simulink model "tractor_mu"  (R2022b)
settings: Solver=FixedStepDiscrete  StartTime=0.0  StopTime=20  FixedStep=0.001  RelTol=1e-3
model workspace (MAT data in the model file):
  P : object (value not decoded)
  w_2 : Simulink.Parameter (value not decoded)
undefined symbols (not defined in the file): A, a, B, b, C, D, DiscIntNeverNeededParam, Iz, K, k1, K1, k2, K2, L1, L2, m, magnitude, Phi, Sample_time, Steer_Ratio
libraries: simulink x26, slpidlib x13, Solver_SF x1, dsparch4 x1
(part 2 of 7)

== system tractor_mu/垂直载荷估算 ==
  ax : Inport
  ay : Inport  Port=2
  roll : Inport  Port=3
  pitch : Inport  Port=4
  MATLAB Function : MATLAB Function  TreatAsAtomicUnit=on
  MATLAB Function1 : MATLAB Function  Commented=on  TreatAsAtomicUnit=on
  MATLAB Function2 : MATLAB Function  Commented=on  TreatAsAtomicUnit=on
  Mux : Mux
  axay : Scope  Commented=on  NumInputPorts=4
  原方法 : Scope  Commented=on  NumInputPorts=4
  Fz1 : Outport
  Fz2 : Outport  Port=2
  Fz3 : Outport  Port=3
  Fz4 : Outport  Port=4
  Fz : Outport  Port=5
  wires:
  ax/1 -> MATLAB Function2/1(ax), MATLAB Function1/1(ax), MATLAB Function/1(ax)
  ay/1 -> MATLAB Function2/2(ay), MATLAB Function1/2(ay), MATLAB Function/2(ay)
  MATLAB Function/2(Fz2) -> Mux/2, Fz2/1
  MATLAB Function/3(Fz3) -> Mux/3, Fz3/1
  MATLAB Function/4(Fz4) -> Mux/4, Fz4/1
  pitch/1 -> MATLAB Function2/3(alpha), MATLAB Function1/3(alpha), MATLAB Function/3(alpha)
  roll/1 -> MATLAB Function2/4(belta), MATLAB Function1/4(belta), MATLAB Function/4(belta)
  MATLAB Function1/1(Fz1) -> axay/1
  MATLAB Function1/2(Fz2) -> axay/2
  MATLAB Function1/3(Fz3) -> axay/3
  MATLAB Function1/4(Fz4) -> axay/4
  MATLAB Function2/1(Fz1) -> 原方法/1
  MATLAB Function2/2(Fz2) -> 原方法/2
  MATLAB Function2/3(Fz3) -> 原方法/3
  MATLAB Function2/4(Fz4) -> 原方法/4
  MATLAB Function/1(Fz1) -> Mux/1, Fz1/1
  Mux/1 -> Fz/1

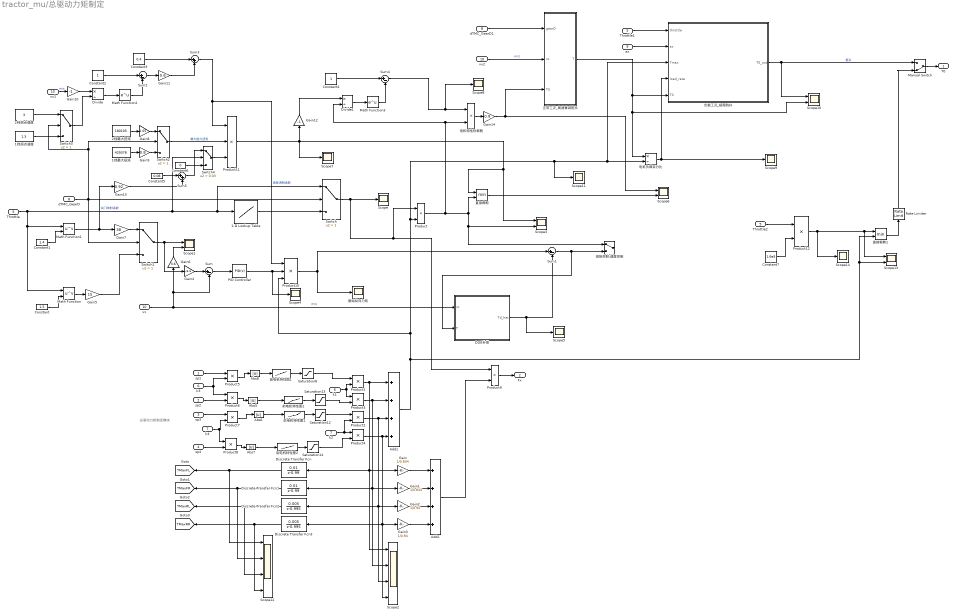
== system tractor_mu/总驱动力矩制定 ==
  note: 总驱动力矩制定模块
  sp1 : Inport
  sp2 : Inport  Port=2
  sp3 : Inport  Port=3
  sp4 : Inport  Port=4
  Throttle : Inport  Port=5
  k1 : Inport  Port=6
  k2 : Inport  Port=7
  dTMC_GearD : Inport  Port=8
  ax : Inport  Port=9
  vx : Inport  Port=10
  1-D Lookup Table : Lookup_n-D  NumberOfTableDimensions=1  BreakpointsForDimension1=[0 0.1 0.2 0.3 0.4 0.5 0.6 0.7 0.8 0.9 1]  Table=[0 0.02 0.04 0.09 0.14 0.23 0.32 0.46 0.6 0.8 1]  InternalRulePriority=Speed  RndMeth=Simplest
  1档拐点速度 : Constant  Value=1.5
  1档最大扭矩 : Constant  Value=429378
  2档拐点速度 : Constant  Value=3
  2档最大扭矩 : Constant  Value=180105
  Abs{5..8} (4 alike) : Abs  SaturateOnIntegerOverflow=off
  Add1 : Sum  Inputs=++++
  Add2 : Sum  Inputs=++++
  Constant : Constant  Value=1.5
  Constant1 : Constant  Value=1.4
  Constant2 : Constant
  Constant3 : Constant  Value=0.4
  Constant4 : Constant
  Constant5 : Constant  Value=0.08
  Constant6 : Constant  Value=0
  Constant7 : Constant  Value=1.6e5
  DOB补偿 : Subsystem
  Discrete Transfer Fcn : DiscreteTransferFcn  Numerator=[0.01]  Denominator=[1 -0.99]
  Discrete Transfer Fcn1 : DiscreteTransferFcn  Numerator=[0.01]  Denominator=[1 -0.99]
  Discrete Transfer Fcn2 : DiscreteTransferFcn  Numerator=[0.005]  Denominator=[1 -0.995]
  Discrete Transfer Fcn3 : DiscreteTransferFcn  Numerator=[0.005]  Denominator=[1 -0.995]
  Divide : Product  Inputs=*/
  Divide1 : Product  Inputs=*/
  Gain : Gain  Gain=1/0.834
  Gain1 : Gain  Gain=1/0.834
  Gain10 : Gain  Gain=-1
  Gain11 : Gain  Gain=0.6
  Gain12 : Gain  Gain=-1
  Gain13 : Gain  Gain=0.92
  Gain14 : Gain  Gain=0.9
  Gain2 : Gain  Gain=1/0.94
  Gain3 : Gain  Gain=1/0.94
  Gain4 : Gain  Gain=1/3.6
  Gain5 : Gain  Gain=15
  Gain6 : Gain  Gain=3.6
  Gain7 : Gain  Gain=38
  Gain8 : Gain  Gain=0.65
  Gain9 : Gain  Gain=0.8
  Manual Switch : ManualSwitch  CurrentSetting=0
  Math Function : Math  Operator=pow
  Math Function1 : Math  Operator=pow
  Math Function2 : Math
  Math Function3 : Math
  PID Controller : slpidlib/PID Controller  Controller=PID  Form=Parallel  TimeDomain=Discrete-time  UseExternalTs=off  SampleTime=-1  IntegratorMethod=Forward Euler  FilterMethod=Forward Euler  ControllerParametersSource=internal  P=0.3  I=0.1  UseKiTs=off  D=0  N=100  UseFilter=on  TunerSelectOption=Transfer Function Based (PID Tuner App)  InitialConditionSource=internal  InitialConditionForIntegrator=0  InitialConditionForFilter=0  DifferentiatorICPrevScaledInput=0  ExternalReset=none  TrackingMode=off  Kt=1  LimitOutput=on  SatLimitsSource=internal  UpperSaturationLimit=1  LowerSaturationLimit=0  LinearizeAsGain=on  AntiWindupMode=none  Kb=1  LimitIntegrator=off  UpperIntegratorSaturationLimit=inf  LowerIntegratorSaturationLimit=-inf  POutMin=[]  POutMax=[]  IOutMin=[]  IOutMax=[]  DOutMin=[]  DOutMax=[]  NOutMin=[]  NOutMax=[]  SumOutMin=[]  SumOutMax=[]  SaturationOutMin=[]  SaturationOutMax=[]  PParamMin=[]  PParamMax=[]  IParamMin=[]  IParamMax=[]  DParamMin=[]  DParamMax=[]  NParamMin=[]  NParamMax=[]  KbParamMin=[]  KbParamMax=[]  KtParamMin=[]  KtParamMax=[]  KbOutMin=[]  KbOutMax=[]  KtOutMin=[]  KtOutMax=[]  IntegratorOutMin=[]  IntegratorOutMax=[]  FilterOutMin=[]  FilterOutMax=[]  SumI1OutMin=[]  SumI1OutMax=[]  SumI2OutMin=[]  SumI2OutMax=[]  SumI3OutMin=[]  SumI3OutMax=[]  SumI4OutMin=[]  SumI4OutMax=[]  SumDOutMin=[]  SumDOutMax=[]  DifferentiatorOutMin=[]  DifferentiatorOutMax=[]  FilterDiffOutCoefMin=[]  FilterDiffOutCoefMax=[]  ReciprocalOutMin=[]  ReciprocalOutMax=[]  SumDenOutMin=[]  SumDenOutMax=[]  SumNumOutMin=[]  SumNumOutMax=[]  DivideOutMin=[]  DivideOutMax=[]  UdiffTsProdOutMin=[]  UdiffTsProdOutMax=[]  NTsProdOutMin=[]  NTsProdOutMax=[]  UintegralTsProdOutMin=[]  UintegralTsProdOutMax=[]  UngainTsProdOutMin=[]  UngainTsProdOutMax=[]  ClampingZeroOutDataTypeStr=Inherit: Inherit via back propagation  ClampingZeroOutMin=[]  ClampingZeroOutMax=[]  FilterDenConstantOutDataTypeStr=Inherit: Inherit via back propagation  FilterDenConstantOutMin=[]  FilterDenConstantOutMax=[]  PCopyOutDataTypeStr=Inherit: Inherit via back propagation  PCopyOutMin=[]  PCopyOutMax=[]  NCopyOutDataTypeStr=Inherit: Inherit via back propagation  NCopyOutMin=[]  NCopyOutMax=[]  IntegratorContinuousStateAttributes=''  IntegratorStateMustResolveToSignalObject=off  IntegratorRTWStateStorageClass=Auto  FilterContinuousStateAttributes=''  FilterStateMustResolveToSignalObject=off  FilterRTWStateStorageClass=Auto  ParallelPVariant=InternalParameters  IdealPVariant=Disabled  IVariant=InternalParameters  DVariant=InternalParameters  IntegratorVariant=Discrete  SatVariant=Enabled  AWVariant=Passthrough  PCopyVariant=Disabled  TRVariant=Disabled  FdbkBlocksVariant=Forward  IdealPFdbkVariant=Disabled  SatFdbkVariant=Disabled  DerivativeFilterVariant=ForwardEulerFilter  NVariant=InternalParameters  NCopyVariant=Disabled  FilterICVariant=InternalICsFilter  IntegratorICVariant=InternalICs  ExternalResetVariant=Disabled  TRSumVariant=Passthrough  SumFdbkVariant=Disabled  SumVariant=Sum_PID  TsampFilterVariant=InternalTs  TsampNgainVariant=Passthrough  TsampIntegralVariant=Passthrough  ExternalSaturationOutDataTypeStr=Inherit: Same as second input
  Product{,1..9,12} (11 alike) : Product
  Product10 : Product  Inputs=3
  Product11 : Product  Inputs=3
  Rate Limiter : RateLimiter  RisingSlewLimit=1.6e5  FallingSlewLimit=-6.4e5  SampleTimeMode=inherited
  Saturation12 : Saturate  UpperLimit=1800  LowerLimit=0
  Saturation13 : Saturate  UpperLimit=1100  LowerLimit=0
  Saturation14 : Saturate  UpperLimit=1800  LowerLimit=0
  Saturation8 : Saturate  UpperLimit=1100  LowerLimit=0
  Scope{,4..5,7..9,11,14} (8 alike) : Scope
  Scope{1,3,6,10,13} (5 alike) : Scope  NumInputPorts=2
  Scope12 : Scope  NumInputPorts=4
  Scope2 : Scope  NumInputPorts=4
  Sum{,1..2,4} (4 alike) : Sum  Inputs=|+-
  Sum3 : Sum  Inputs=|++
  Sum5 : Sum  Inputs=|++
  Switch{,1..3} (4 alike) : Switch  Criteria=u2 > Threshold  Threshold=1  SaturateOnIntegerOverflow=off  InputSameDT=off
  Switch4 : Switch  Criteria=u2 > Threshold  Threshold=0.03  SaturateOnIntegerOverflow=off  InputSameDT=off
  Throttle1 : InportShadow  Port=5
  Throttle2 : InportShadow  Port=5
  dTMC_GearD1 : InportShadow  Port=8
  k3 : InportShadow  Port=6
  k4 : InportShadow  Port=7
  vx1 : InportShadow  Port=10
  vx2 : InportShadow  Port=10
  前电机特性图1 : Lookup_n-D  NumberOfTableDimensions=1  BreakpointsForDimension1=[0;600;900;1200;1500;1800;2104;2402;2701;3001;3302;3600;3901;4200;4501;4801;5000;5001]  Table=[1116;1107;1102;1099;1101;913;734;611;523;456;403;363;327;305;278;253;240;0]  InternalRulePriority=Speed  OutMin=0  OutMax=1200  RndMeth=Simplest
  前电机特性图2 : Lookup_n-D  NumberOfTableDimensions=1  BreakpointsForDimension1=[0;600;900;1200;1500;1800;2104;2402;2701;3001;3302;3600;3901;4200;4501;4801;5000;5001]  Table=[1116;1107;1102;1099;1101;913;734;611;523;456;403;363;327;305;278;253;240;0]  InternalRulePriority=Speed  OutMin=0  OutMax=1200  RndMeth=Simplest
  原始纵向力矩 : Scope
  后电机特性图1 : Lookup_n-D  NumberOfTableDimensions=1  BreakpointsForDimension1=[0;299;599.6;899.7;1200;1500;1800;2099;2399.4;2698.5;2998.1;3300;3599;3899;4197.8;4201]  Table=[1868;1868.3;1868.6;1844.3;1842.3;1763.9;1516.4;1277.9;1098.6;954;839.4;727;645.7;585.53;529.7;0]  InternalRulePriority=Speed  OutMin=[0]  OutMax=[1800]  RndMeth=Simplest
  后电机特性图2 : Lookup_n-D  NumberOfTableDimensions=1  BreakpointsForDimension1=[0;500;1000;1200;1600;2000;2800;3200;3600;4200;4201]  Table=[1800;1800;1800;1800;1700;1360;900;750;650;520;0]  InternalRulePriority=Speed  OutMin=[0]  OutMax=[1800]  RndMeth=Simplest
  扭矩控制/速度控制 : ManualSwitch
  正常工况_高速衰减防抖 : Subsystem
  电机特性软裁剪 : Product
  电机负载百分比 : Product  Inputs=*/
  直接裁剪 : MinMax  Inputs=2
  直接裁剪1 : MinMax  Inputs=2
  负载工况_极限防抖 : Stateflow chart  TreatAsAtomicUnit=on
  T0 : Outport
  Fx : Outport  Port=2
  tag scope: TMaxFL=global, TMaxFR=global, TMaxRL=global, TMaxRR=global
  wires:
  sp3/1 -> Product7/1
  Saturation8/1 -> Product1/1
  前电机特性图2/1 -> Saturation13/1
  后电机特性图1/1 -> Saturation12/1
  sp1/1 -> Product5/1
  sp4/1 -> Product8/2
  Abs7/1 -> 后电机特性图2/1
  Product2/1 -> Discrete Transfer Fcn2/1, Scope2/3, Gain2/1, Add1/3
  前电机特性图1/1 -> Saturation8/1
  sp2/1 -> Product6/2
  Product3/1 -> Add1/2, Discrete Transfer Fcn1/1, Scope2/2, Gain1/1
  后电机特性图2/1 -> Saturation14/1
  Saturation12/1 -> Product2/1
  Abs5/1 -> 前电机特性图2/1
  Abs6/1 -> 后电机特性图1/1
  Abs8/1 -> 前电机特性图1/1
  k1/1 -> Product3/1, Product1/2
  Saturation13/1 -> Product3/2
  k2/1 -> Product4/1, Product2/2
  Saturation14/1 -> Product4/2
  Product4/1 -> Discrete Transfer Fcn3/1, Scope2/4, Gain3/1, Add1/4
  Product/1 -> Divide1/2, 电机特性软裁剪/2, 直接裁剪/2, Scope3/2, 扭矩控制/速度控制/1
  k3/1 -> Product6/1, Product5/2
  Product5/1 -> Abs8/1
  Product6/1 -> Abs5/1
  k4/1 -> Product8/1, Product7/2
  Product7/1 -> Abs6/1
  Product8/1 -> Abs7/1
  1-D Lookup Table/1 -> Switch/3
  Gain/1 -> Add2/1
  Gain1/1 -> Add2/2
  Gain2/1 -> Add2/3
  Gain3/1 -> Add2/4
  Add2/1 -> Product9/2
  Product9/1 -> Fx/1
  Throttle/1 -> Math Function/1, Math Function1/1, Switch4/2, Switch/1, 1-D Lookup Table/1
  Constant/1 -> Math Function/2
  Math Function/1 -> Gain5/1
  Gain5/1 -> Switch1/3
  Constant1/1 -> Math Function1/2
  Gain7/1 -> Switch1/1
  Math Function1/1 -> Gain13/1, Gain7/1  "油门映射函数"
  Switch1/1 -> Gain4/1, Scope1/1
  Gain4/1 -> Sum/1
  vx/1 -> Sum/2, Gain6/1, DOB补偿/1(vx)  "m/s"
  Switch/1 -> Product9/1, Product/1, Scope/1
  Sum/1 -> PID Controller/1
  PID Controller/1 -> Scope4/1, Product10/2
  Product10/1 -> Sum1/1, 原始纵向力矩/1
  Gain6/1 -> Scope1/2
  Sum1/1 -> DOB补偿/2(T), 扭矩控制/速度控制/2
  DOB补偿/1(Td_hat) -> Scope5/1, Sum1/2
  1档最大扭矩/1 -> Gain9/1
  2档最大扭矩/1 -> Gain8/1
  Gain8/1 -> Switch2/1
  Gain9/1 -> Switch2/3
  Switch2/1 -> Product11/2  "最大能力扭矩"
  Constant2/1 -> Sum2/1
  Math Function2/1 -> Sum2/2
  1档拐点速度/1 -> Switch3/3
  2档拐点速度/1 -> Switch3/1
  dTMC_GearD/1 -> Switch3/2, Switch2/2, Switch1/2, Switch/2
  vx1/1 -> Gain10/1  "m/s"
  Switch3/1 -> Divide/2
  Gain10/1 -> Divide/1
  Divide/1 -> Math Function2/1
  Sum2/1 -> Gain11/1
  Constant3/1 -> Sum3/1
  Gain11/1 -> Sum3/2
  Sum3/1 -> Product10/1, Product11/1  "速度调制函数"
  Constant4/1 -> Sum4/1
  Math Function3/1 -> Sum4/2
  Divide1/1 -> Math Function3/1
  Gain12/1 -> Divide1/1
  Sum4/1 -> Scope8/1, 电机特性软裁剪/1
  Product11/1 -> Scope7/1, 直接裁剪/1, Scope3/1, Gain12/1
  Sum5/1 -> Switch4/1
  Gain13/1 -> Sum5/2
  Constant5/1 -> Sum5/1
  Switch4/1 -> Product11/3
  Constant6/1 -> Switch4/3
  电机特性软裁剪/1 -> Gain14/1
  直接裁剪/1 -> Scope6/2
  Product1/1 -> Discrete Transfer Fcn/1, Scope2/1, Gain/1, Add1/1
  dTMC_GearD1/1 -> 正常工况_高速衰减防抖/1(gearD)
  vx2/1 -> 正常工况_高速衰减防抖/2(vx)  "m/s"
  Throttle1/1 -> 负载工况_极限防抖/1(throttle)
  ax/1 -> 负载工况_极限防抖/2(ax)
  Add1/1 -> Scope13/2, 直接裁剪1/2, Scope11/1, 负载工况_极限防抖/3(Tmax), 电机负载百分比/2, Product/2, Product10/3
  正常工况_高速衰减防抖/1(T) -> 负载工况_极限防抖/5(T0), Scope10/2, 电机负载百分比/1
  电机负载百分比/1 -> 负载工况_极限防抖/4(load_rate), Scope9/1
  负载工况_极限防抖/1(T0_out) -> Manual Switch/1, Scope10/1  "复杂"
  Discrete Transfer Fcn/1 -> Scope12/1, [TMaxFL]
  Discrete Transfer Fcn1/1 -> Scope12/2, [TMaxFR]
  Discrete Transfer Fcn2/1 -> Scope12/3, [TMaxRL]
  Discrete Transfer Fcn3/1 -> Scope12/4, [TMaxRR]
  Gain14/1 -> Scope6/1, 正常工况_高速衰减防抖/3(T0)
  Manual Switch/1 -> T0/1
  Throttle2/1 -> Product12/1
  Constant7/1 -> Product12/2
  Product12/1 -> Scope13/1, 直接裁剪1/1, Scope14/1
  直接裁剪1/1 -> Rate Limiter/1
  Rate Limiter/1 -> Manual Switch/2

== system tractor_mu/挡位与刹车处理1 ==
  dTMC_GearD : Inport
  Constant6 : Constant  Value=15.88
  Constant7 : Constant  Value=30.6204
  Constant8 : Constant  Value=63.52
  Constant9 : Constant  Value=80.454
  Switch2 : Switch  Criteria=u2 > Threshold  Threshold=1  SaturateOnIntegerOverflow=off  InputSameDT=off
  Switch3 : Switch  Criteria=u2 > Threshold  Threshold=1  SaturateOnIntegerOverflow=off  InputSameDT=off
  spdratio_F : Outport
  spdratio_R : Outport  Port=2
  wires:
  Switch3/1 -> spdratio_R/1
  Constant9/1 -> Switch3/3
  Switch2/1 -> spdratio_F/1
  Constant8/1 -> Switch2/3
  dTMC_GearD/1 -> Switch3/2, Switch2/2
  Constant6/1 -> Switch2/1
  Constant7/1 -> Switch3/1

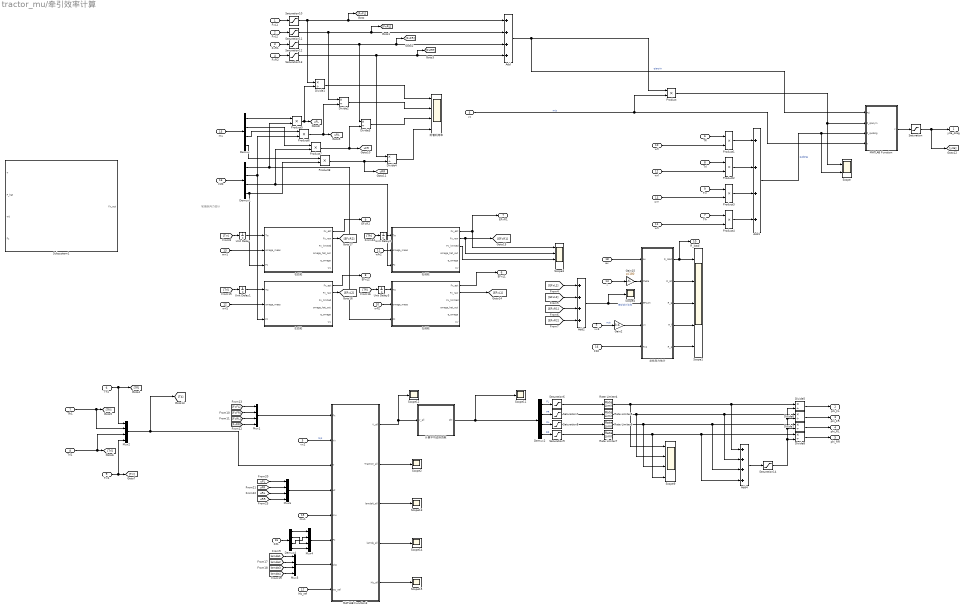
== system tractor_mu/牵引效率计算 ==
  note: 轮端纵向力估计
  FxL1 : Inport
  FxL2 : Inport  Port=2
  FxR1 : Inport  Port=3
  FxR2 : Inport  Port=4
  vx : Inport  Port=5
  Tfl : Inport  Port=6
  Tfr : Inport  Port=7
  Trl : Inport  Port=8
  Trr : Inport  Port=9
  wfl : Inport  Port=10
  wfr : Inport  Port=11
  wrl : Inport  Port=12
  wrr : Inport  Port=13
  i : Inport  Port=14
  mu : Inport  Port=15
  FZ0 : Inport  Port=16
  Mz_ref : Inport  Port=17
  ax : Inport  Port=18
  Add{,1..2,4} (4 alike) : Sum  Inputs=++++
  Demux{,1..2,4} (4 alike) : Demux
  Divide{1..8} (8 alike) : Product  Inputs=*/
  FZ1 : InportShadow  Port=16
  FZ2 : InportShadow  Port=16
  Gain15 : Gain  Gain=pi/180
  Gain2 : Gain  Gain=3.6
  MATLAB Function : MATLAB Function  TreatAsAtomicUnit=on
  MATLAB Function3 : MATLAB Function  TreatAsAtomicUnit=on
  Mux{1..2,4..6} (5 alike) : Mux
  Product{,1..8} (9 alike) : Product
  Rate Limiter{4..7} (4 alike) : RateLimiter  RisingSlewLimit=2e5  FallingSlewLimit=-2e5  SampleTimeMode=inherited
  Saturation : Saturate  UpperLimit=999  LowerLimit=-999
  Saturation{6..13} (8 alike) : Saturate  UpperLimit=99999999  LowerLimit=0
  Saturation14 : Saturate  UpperLimit=99999999999999  LowerLimit=0.01
  Scope : Scope  NumInputPorts=2
  Scope1 : Scope  NumInputPorts=5
  Scope{2,4,11..15} (7 alike) : Scope
  Scope3 : Scope  NumInputPorts=4
  Scope9 : Scope  NumInputPorts=4
  Subsystem1 : Subsystem
  Tfl1 : InportShadow  Port=6
  Tfr1 : InportShadow  Port=7
  Trl1 : InportShadow  Port=8
  Trr1 : InportShadow  Port=9
  Unit Delay{,1..3} (4 alike) : UnitDelay  SampleTime=-1  HasFrameUpgradeWarning=on
  mu1 : InportShadow  Port=15
  vx2 : InportShadow  Port=5
  vx3 : InportShadow  Port=5
  wfl2 : InportShadow  Port=10
  wfr2 : InportShadow  Port=11
  wrl1 : InportShadow  Port=12
  wrr1 : InportShadow  Port=13
  右前轮 : MATLAB Function  TreatAsAtomicUnit=on
  右后轮 : MATLAB Function  TreatAsAtomicUnit=on
  左前轮 : MATLAB Function  TreatAsAtomicUnit=on
  左后轮 : MATLAB Function  TreatAsAtomicUnit=on
  总纵向力估计 : Subsystem
  计算平均边际贡献 : MATLAB Function  TreatAsAtomicUnit=on
  附着利用率 : Scope  NumInputPorts=4
  yita_drag : Outport
  phi_FL : Outport  Port=2
  phi_FR : Outport  Port=3
  phi_RL : Outport  Port=4
  phi_RR : Outport  Port=5
  EFxL1 : Outport  Port=6
  EFxR1 : Outport  Port=7
  EFxL2 : Outport  Port=8
  EFxR2 : Outport  Port=9
  R_load : Outport  Port=10
  tag scope: uFL=global, uFR=global, uRL=global, uRR=global
  wires:
  FxR2/1 -> Saturation13/1
  FxR1/1 -> Saturation12/1
  FxL2/1 -> Saturation11/1
  FxL1/1 -> Saturation10/1
  Tfl/1 -> Product1/1
  wfl/1 -> Product1/2
  Trl/1 -> Product2/1
  Trr/1 -> Product3/1
  wrr/1 -> Product3/2
  wrl/1 -> Product2/2
  wfr/1 -> Product4/2
  Tfr/1 -> Product4/1
  Product4/1 -> Add1/4
  Product3/1 -> Add1/3
  Product2/1 -> Add1/2
  Product1/1 -> Add1/1
  Add1/1 -> MATLAB Function/3(P_qudong), Scope/2  "qudong"
  MATLAB Function/1(y) -> Saturation/1
  Add/1 -> Product/1, MATLAB Function/1(Fd)  "qianyin"
  vx/1 -> MATLAB Function/4(v), Product/2  "m/s"
  Product/1 -> MATLAB Function/2(P_qianyin), Scope/1
  mu/1 -> Demux/1
  FZ0/1 -> Demux1/1
  Demux/1 -> Product5/1
  Product5/1 -> [uFL], Divide1/2
  Demux/2 -> Product7/1
  Product6/1 -> [uRL], Divide2/2
  Demux/3 -> Product6/1
  Demux/4 -> Product8/1
  Product7/1 -> [uFR], Divide3/2
  Product8/1 -> [uRR], Divide4/2
  Saturation/1 -> [yita], yita_drag/1
  Divide2/1 -> 附着利用率/2
  Divide1/1 -> 附着利用率/1
  Divide4/1 -> 附着利用率/4
  Divide3/1 -> 附着利用率/3
  计算平均边际贡献/1(phi) -> Demux2/1, Scope11/1
  Demux2/2 -> Saturation7/1  "FR"
  Demux2/1 -> Saturation6/1  "FL"
  Demux2/3 -> Saturation8/1  "RL"
  Demux2/4 -> Saturation9/1  "RR"
  Rate Limiter4/1 -> Scope9/1, Divide5/1, Add4/1
  Rate Limiter5/1 -> Scope9/2, Add4/2, Divide6/1
  Rate Limiter6/1 -> Scope9/3, Divide7/1, Add4/3
  Add4/1 -> Saturation14/1
  Divide5/1 -> phi_FL/1
  Divide6/1 -> phi_FR/1
  Divide7/1 -> phi_RL/1
  Divide8/1 -> phi_RR/1
  Mux1/1 -> MATLAB Function3/1(Fx)
  vx2/1 -> MATLAB Function3/2(Vx)  "m/s"
  Tfl1/1 -> [Tfl], Mux2/1
  Tfr1/1 -> [Tfr], Mux2/2
  Trr1/1 -> [Trr], Mux2/4
  mu1/1 -> MATLAB Function3/5(mu)
  FZ1/1 -> Demux4/1
  Demux4/1 -> Mux4/1
  Demux4/4 -> Mux4/4
  Demux4/2 -> Mux4/3
  Demux4/3 -> Mux4/2
  Mux4/1 -> MATLAB Function3/6(Fz)
  Mz_ref/1 -> MATLAB Function3/8(Mz_ref)
  MATLAB Function3/1(V_all) -> Scope12/1, 计算平均边际贡献/1(v_all)
  MATLAB Function3/2(Traction_all) -> Scope2/1
  MATLAB Function3/3(lamdaN_all) -> Scope13/1
  MATLAB Function3/4(lamda_all) -> Scope14/1
  MATLAB Function3/5(Mz_all) -> Scope15/1
  Saturation10/1 -> [FxFL], Add/1, Divide1/1
  Saturation11/1 -> [FxRL], Add/2, Divide2/1
  Saturation12/1 -> [FxFR], Add/3, Divide3/1
  Saturation13/1 -> [FxRR], Add/4, Divide4/1
  Saturation6/1 -> Rate Limiter4/1
  Saturation7/1 -> Rate Limiter5/1
  Saturation8/1 -> Rate Limiter6/1
  Saturation9/1 -> Rate Limiter7/1
  Rate Limiter7/1 -> Scope9/4, Add4/4, Divide8/1
  Saturation14/1 -> Divide8/2, Divide7/2, Divide6/2, Divide5/2
  Mux5/1 -> MATLAB Function3/7(slip)
  [lamda1] -> Mux5/1
  [lamda2] -> Mux5/2
  [lamda3] -> Mux5/3
  [lamda4] -> Mux5/4
  [uRR] -> Mux6/4
  [uRL] -> Mux6/3
  [uFR] -> Mux6/2
  [uFL] -> Mux6/1
  Mux6/1 -> MATLAB Function3/4(uF)
  [FxRR] -> Mux1/4
  [FxRL] -> Mux1/3
  [FxFR] -> Mux1/2
  [FxFL] -> Mux1/1
  ax/1 -> 总纵向力估计/1(ax)
  Mux2/1 -> [T4], MATLAB Function3/3(T)
  vx3/1 -> Gain2/1  "m/s"
  Gain2/1 -> 总纵向力估计/4(vx)
  Gain15/1 -> 总纵向力估计/2(theta)
  Demux1/1 -> 左前轮/3(Fz), Product5/2
  wrl1/1 -> 左后轮/2(omega_meas)
  wrr1/1 -> 右后轮/2(omega_meas)
  Demux1/3 -> 右前轮/3(Fz), Product7/2
  Demux1/2 -> Product6/2, 左后轮/3(Fz)
  Demux1/4 -> 右后轮/3(Fz), Product8/2
  Trl1/1 -> [Trl], Mux2/3
  i/1 -> Gain15/1
  [EFxL1] -> Add2/1
  [EFxL2] -> Add2/2
  [EFxR1] -> Add2/3
  [EFxR2] -> Add2/4
  Add2/1 -> Scope4/1, 总纵向力估计/3(EFsum)  "单轮估计总和"
  [Trr] -> Unit Delay/1
  [Trl] -> Unit Delay1/1
  [Tfl] -> Unit Delay3/1
  [Tfr] -> Unit Delay2/1
  wfl2/1 -> 左前轮/2(omega_meas)
  wfr2/1 -> 右前轮/2(omega_meas)
  左前轮/1(Fx_est) -> EFxL1/1
  右前轮/1(Fx_est) -> Scope3/1, EFxR1/1
  左后轮/1(Fx_est) -> EFxL2/1
  右后轮/1(Fx_est) -> EFxR2/1
  FZ2/1 -> 总纵向力估计/5(Fz4)
  总纵向力估计/1(R_load) -> R_load/1, Scope1/1
  总纵向力估计/2(R_all) -> Scope1/2
  总纵向力估计/3(R_g) -> Scope1/3
  总纵向力估计/4(R_f) -> Scope1/4
  总纵向力估计/5(R_a) -> Scope1/5
  右前轮/2(Fx_raw) -> [EFxR1], Scope3/2
  右前轮/3(Fx_limited) -> Scope3/3
  右后轮/2(Fx_raw) -> [EFxR2]
  左后轮/2(Fx_raw) -> [EFxL2]
  左前轮/2(Fx_raw) -> [EFxL1]
  Unit Delay/1 -> 右后轮/1(Tw)
  Unit Delay1/1 -> 左后轮/1(Tw)
  Unit Delay2/1 -> 右前轮/1(Tw)
  Unit Delay3/1 -> 左前轮/1(Tw)

== system tractor_mu/质心侧偏角估计 ==
  Steer_L1_Carsim : Inport
  Ay_Carsim : Inport  Port=2
  Avz_Carsim : Inport  Port=3
  vx : Inport  Port=4
  Constant : Constant  Commented=on  Value=A
  Constant1 : Constant  Commented=on  Value=B
  Constant2 : Constant  Commented=on  Value=C
  Constant3 : Constant  Commented=on  Value=D
  Constant4 : Constant  Commented=on  Value=C
  Constant5 : Constant  Commented=on  Value=D
  Constant6 : Constant  Value=0
  Constant7 : Constant  Value=0.001  OutDataTypeStr=single
  Data Type Conversion{,2..4} (4 alike) : DataTypeConversion  OutDataTypeStr=single  SaturateOnIntegerOverflow=off  RndMeth=Floor
  Demux : Demux  Outputs=2
  From6 : From
  Gain : Gain
  Goto3 : Goto
  Kalman Filter : Subsystem
  Mux : Mux  Inputs=2
  Observer : Subsystem
  Signal Specification : SignalSpecification  OutDataTypeStr=single
  Terminator : Terminator
  Unit Delay : UnitDelay  SampleTime=-1  HasFrameUpgradeWarning=on
  define_Kalman : MATLAB Function  TreatAsAtomicUnit=on
  Beta_estimate_3 : Outport
  wires:
  Steer_L1_Carsim/1 -> [Steer_L1]
  Ay_Carsim/1 -> Mux/1
  Avz_Carsim/1 -> Mux/2
  Mux/1 -> [y]
  [Steer_L1] -> Observer/1(u[k])
  [y] -> Observer/2(y[k])
  Observer/1(x[k+1|k]) -> Unit Delay/1
  Unit Delay/1 -> [xhat]
  [xhat] -> Observer/8(xhat[k|k-1])
  [Steer_L1] -> Kalman Filter/1(u[k])
  [y] -> Kalman Filter/2(y[k])
  [xhat] -> Kalman Filter/5(xhat[k|k-1])
  Demux/1 -> Gain/1
  Demux/2 -> Terminator/1
  Constant6/1 -> Observer/7(L[k])
  vx/1 -> Data Type Conversion3/1
  define_Kalman/1(A) -> Goto3/1
  define_Kalman/2(B) -> [B]
  define_Kalman/3(C) -> [C]
  define_Kalman/4(D) -> [D]
  From6/1 -> Observer/3(A[k])
  [B] -> Observer/4(B[k])
  [C] -> Observer/5(C[k])
  [D] -> Observer/6(D[k])
  [C] -> Kalman Filter/3(C[k])
  [D] -> Kalman Filter/4(D[k])
  Constant7/1 -> Kalman Filter/12(Sample_time)
  define_Kalman/10(c12) -> Signal Specification/1
  define_Kalman/9(c11) -> Data Type Conversion/1
  define_Kalman/8(a22) -> Data Type Conversion2/1
  define_Kalman/6(a12) -> Kalman Filter/7(a12)
  define_Kalman/5(a11) -> Kalman Filter/6(a11)
  Signal Specification/1 -> Kalman Filter/11(c12)
  Data Type Conversion3/1 -> define_Kalman/1(u)
  define_Kalman/7(a21) -> Data Type Conversion4/1
  Data Type Conversion2/1 -> Kalman Filter/9(a22)
  Data Type Conversion/1 -> Kalman Filter/10(c11)
  Kalman Filter/1(xhat[k|k]) -> Demux/1
  Data Type Conversion4/1 -> Kalman Filter/8(a21)
  Gain/1 -> Beta_estimate_3/1  "beta"

== system tractor_mu/质心侧偏角滑模观测器估计 ==
  Steer_L1_Carsim : Inport
  Avz_Carsim : Inport  Port=2
  vx : Inport  Port=3
  Subsystem : Subsystem
      settings: PortSchema="{\"entries\":[{\"content\":{\"sides\":[{\"content\":{\"connectorIds\":[\"In1\",\"In2\"]},\"type\":\"ConnectorPlacement.EquallySpacedRectSide\",\"uuid\":\"f261e0cd-ec93-4f62-a19f-443007200df0\"},{\"content\":{\"connectorIds\":[\"Out1\",\"Out2\",\"Out3\"],\"side\":\"RIGHT\"},\"type\":\"ConnectorPlacement.EquallySpacedRectSide\",\"uuid\":\"f7fa71f6-b20e-403a-8d6a-a83336d9dad7\"},{\"content\":{\"side\":\"TOP\"},\"type\":\"ConnectorPlacement.EquallySpacedRectSide\",\"uuid\":\"43a2f696-43ec-479c-b2ef-38a272620956\"},{\"content\":{\"connectorIds\":[\"In3\"],\"side\":\"BOTTOM\"},\"type\":\"ConnectorPlacement.EquallySpacedRectSide\",\"uuid\":\"cccb66fe-f25e-4bdd-bd00-f2c86639dcdc\"}]},\"type\":\"ConnectorPlacement.EquallySpacedConnector\",\"uuid\":\"c7d73279-bbf7-49af-a87e-cb8836bffa13\"}],\"packageUris\":[\"http://schema.mathworks.com/mf0/Connector/R2020b\"],\"version\":\"1.0\"}"
  Subsystem1 : Subsystem  Commented=on
      settings: PortSchema="{\"entries\":[{\"content\":{\"sides\":[{\"content\":{\"connectorIds\":[\"In1\",\"In2\"]},\"type\":\"ConnectorPlacement.EquallySpacedRectSide\",\"uuid\":\"f261e0cd-ec93-4f62-a19f-443007200df0\"},{\"content\":{\"connectorIds\":[\"Out1\",\"Out2\",\"Out3\"],\"side\":\"RIGHT\"},\"type\":\"ConnectorPlacement.EquallySpacedRectSide\",\"uuid\":\"f7fa71f6-b20e-403a-8d6a-a83336d9dad7\"},{\"content\":{\"side\":\"TOP\"},\"type\":\"ConnectorPlacement.EquallySpacedRectSide\",\"uuid\":\"43a2f696-43ec-479c-b2ef-38a272620956\"},{\"content\":{\"connectorIds\":[\"In3\"],\"side\":\"BOTTOM\"},\"type\":\"ConnectorPlacement.EquallySpacedRectSide\",\"uuid\":\"cccb66fe-f25e-4bdd-bd00-f2c86639dcdc\"}]},\"type\":\"ConnectorPlacement.EquallySpacedConnector\",\"uuid\":\"c7d73279-bbf7-49af-a87e-cb8836bffa13\"}],\"packageUris\":[\"http://schema.mathworks.com/mf0/Connector/R2020b\"],\"version\":\"1.0\"}"
  delta_f : Gain  Gain=1/Steer_Ratio
  beta_est : Outport
  gamma_est : Outport  Port=2
  vy_hat_out : Outport  Port=3
  wires:
  Steer_L1_Carsim/1 -> delta_f/1
  Avz_Carsim/1 -> Subsystem/1(Avz_Carsim)
  vx/1 -> Subsystem/2(vx)
  delta_f/1 -> Subsystem/3(delta_f)
  Subsystem/1(beta_est) -> beta_est/1
  Subsystem/2(gamma_est) -> gamma_est/1
  Subsystem/3(vy_hat_output) -> vy_hat_out/1

== system tractor_mu/质心侧偏角观测 ==
  前轮转角 : Inport
  前轮纵向力 : Inport  Port=2
  后轮纵向力 : Inport  Port=3
  纵向速度 : Inport  Port=4
  横摆角速度 : Inport  Port=5
  Demux : Demux  Outputs=3
  Gain : Gain  Gain=0.001
  MATLAB Function : MATLAB Function  TreatAsAtomicUnit=on
  Mux : Mux  Inputs=3
  Mux1 : Mux  Inputs=2
  Scope : Scope
  Scope1 : Scope
  Sum : Sum  Inputs=|++
  Sum1 : Sum  Inputs=|+-
  Unit Delay : UnitDelay  InitialCondition=[0.1;0;0]  SampleTime=0.001  HasFrameUpgradeWarning=on
  Unit Delay1 : UnitDelay  InitialCondition=[0.1;0;0]  SampleTime=0.001  HasFrameUpgradeWarning=on
  估计横摆角速度 : Scope
  估计纵向速度 : Scope
  侧偏角估计 : Scope
  侧偏角 : Outport
  纵向速度估计 : Outport  Port=2
  横摆角速度估计 : Outport  Port=3
  wires:
  MATLAB Function/1(x_dot) -> Scope1/1, Gain/1
  Gain/1 -> Sum/1
  Unit Delay/1 -> Sum/2
  Sum/1 -> Unit Delay1/1, Demux/1, Unit Delay/1
  Demux/2 -> 侧偏角估计/1, 侧偏角/1
  Demux/1 -> 纵向速度估计/1, 估计纵向速度/1
  Demux/3 -> 横摆角速度估计/1, 估计横摆角速度/1
  前轮转角/1 -> Mux/1
  前轮纵向力/1 -> Mux/2
  后轮纵向力/1 -> Mux/3
  Mux/1 -> MATLAB Function/2(u)
  纵向速度/1 -> Mux1/1
  横摆角速度/1 -> Mux1/2
  Mux1/1 -> Sum1/1, MATLAB Function/3(z_meas)
  MATLAB Function/2(z_hat) -> Sum1/2
  Sum1/1 -> Scope/1
  Unit Delay1/1 -> MATLAB Function/1(x_hat)

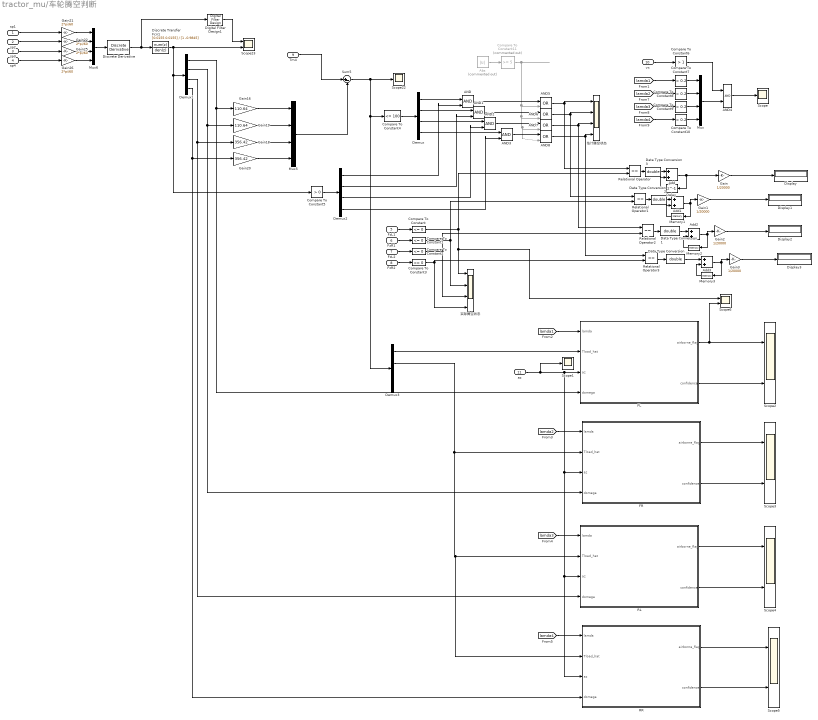
== system tractor_mu/车轮腾空判断 ==
  sp1 : Inport
  sp2 : Inport  Port=2
  sp3 : Inport  Port=3
  sp4 : Inport  Port=4
  FzL1 : Inport  Port=5
  FzR1 : Inport  Port=6
  FzL2 : Inport  Port=7
  FzR2 : Inport  Port=8
  Tm4 : Inport  Port=9
  vx : Inport  Port=10
  az : Inport  Port=11
  AND{,1..4} (5 alike) : Logic  IconShape=distinctive  AllPortsSameDT=off  OutDataTypeStr=boolean
  AND{5..8} (4 alike) : Logic  Operator=OR  IconShape=distinctive  AllPortsSameDT=off  OutDataTypeStr=boolean
  Abs : Abs  Commented=on  SaturateOnIntegerOverflow=off
  Add : Sum
  Add1 : Sum
  Add2 : Sum
  Add3 : Sum  AccumDataTypeStr=double
  Compare To Constant{,1..3} (4 alike) : simulink/Logic and Bit Operations/Compare To Constant  relop=<=  const=0  OutDataTypeStr=boolean
  Compare To Constant{7..10} (4 alike) : simulink/Logic and Bit Operations/Compare To Constant  relop=>  const=0.2  OutDataTypeStr=boolean
  Compare To Constant11 : simulink/Logic and Bit Operations/Compare To Constant  Commented=on  relop=>=  const=5  OutDataTypeStr=boolean
  Compare To Constant4 : simulink/Logic and Bit Operations/Compare To Constant  relop=<=  const=100  OutDataTypeStr=boolean
  Compare To Constant5 : simulink/Logic and Bit Operations/Compare To Constant  relop=>  const=0  OutDataTypeStr=boolean
  Compare To Constant6 : simulink/Logic and Bit Operations/Compare To Constant  relop=>  const=1  OutDataTypeStr=boolean
  Data Type Conversion{,1..3} (4 alike) : DataTypeConversion  OutDataTypeStr=double  SaturateOnIntegerOverflow=off  RndMeth=Floor
  Delay : Delay  DelayLength=1
  Demux{,1..3} (4 alike) : Demux
  Digital Filter Design1 : dsparch4/Digital Filter Design  mwdsp_browser_bugfix_var=off
  Discrete Transfer Fcn1 : DiscreteTransferFcn  Numerator=[0.0155 0.0155]  Denominator=[1 -0.9845]
  Discrete Derivative : simulink/Discrete/Discrete Derivative  gainval=1.0  ICPrevScaledInput=0.0  OutMin=[]  OutMax=[]  OutDataType=fixdt(1, 16)  OutScaling=2^-10  DoSatur=off
  Display{,1..3} (4 alike) : Display
  FL : Stateflow chart  TreatAsAtomicUnit=on
  FR : Stateflow chart  TreatAsAtomicUnit=on
  Gain{,1..3} (4 alike) : Gain  Gain=1/20000
  Gain16 : Gain  Gain=110.64
  Gain18 : Gain  Gain=356.42
  Gain19 : Gain  Gain=110.64
  Gain20 : Gain  Gain=356.42
  Gain{21..22,25..26} (4 alike) : Gain  Gain=2*pi/60
  Memory1 : Memory
  Memory2 : Memory
  Memory3 : Memory
  Mux : Mux
  Mux5 : Mux
  Mux6 : Mux
  RL : Stateflow chart  TreatAsAtomicUnit=on
  RR : Stateflow chart  TreatAsAtomicUnit=on
  Relational Operator{,1..3} (4 alike) : RelationalOperator  Operator===  OutDataTypeStr=boolean  RndMeth=Simplest  InputSameDT=off
  Scope : Scope
  Scope1 : Scope
  Scope{2..6,23} (6 alike) : Scope  NumInputPorts=2
  Scope22 : Scope
  Sum5 : Sum  Inputs=|+-
  估计腾空状态 : Scope  NumInputPorts=4
  实际腾空状态 : Scope  NumInputPorts=4
  wires:
  Digital Filter Design1/1 -> Scope23/1
  Compare To Constant2/1 -> Relational Operator2/2, 实际腾空状态/3
  sp2/1 -> Gain22/1
  Discrete Transfer Fcn1/1 -> Compare To Constant5/1, Demux1/1, Scope23/2
  Compare To Constant3/1 -> Relational Operator3/2, 实际腾空状态/4
  Compare To Constant/1 -> Relational Operator/2, Scope6/1, 实际腾空状态/1
  FzL1/1 -> Compare To Constant/1
  Gain21/1 -> Mux6/1
  Mux5/1 -> Sum5/2
  Tm4/1 -> Sum5/1
  Mux6/1 -> Discrete Derivative/1
  Gain19/1 -> Mux5/2
  Gain26/1 -> Mux6/4
  Discrete Derivative/1 -> Digital Filter Design1/1, Discrete Transfer Fcn1/1
  Gain22/1 -> Mux6/2
  Compare To Constant1/1 -> Relational Operator1/2, 实际腾空状态/2
  Gain18/1 -> Mux5/3
  Gain25/1 -> Mux6/3
  Gain20/1 -> Mux5/4
  FzR2/1 -> Compare To Constant3/1
  Demux1/1 -> FL/4(domega), Gain16/1
  FzL2/1 -> Compare To Constant2/1
  Gain16/1 -> Mux5/1
  FzR1/1 -> Compare To Constant1/1
  sp4/1 -> Gain26/1
  sp1/1 -> Gain21/1
  sp3/1 -> Gain25/1
  Compare To Constant4/1 -> Demux/1
  Compare To Constant5/1 -> Demux2/1
  Demux/1 -> AND/1
  Demux2/1 -> AND/2
  Demux/2 -> AND1/1
  Demux2/2 -> AND1/2
  Demux/3 -> AND2/1
  Demux2/3 -> AND2/2
  Demux/4 -> AND3/1
  Demux2/4 -> AND3/2
  AND8/1 -> 估计腾空状态/4, Relational Operator3/1
  AND7/1 -> 估计腾空状态/3, Relational Operator2/1
  AND6/1 -> 估计腾空状态/2, Relational Operator1/1
  AND5/1 -> 估计腾空状态/1, Relational Operator/1
  Relational Operator/1 -> Data Type Conversion3/1
  Gain/1 -> Display/1
  Gain1/1 -> Display1/1
  Gain2/1 -> Display2/1
  Gain3/1 -> Display3/1
  Add/1 -> Delay/1, Gain/1
  Delay/1 -> Add/2
  Relational Operator1/1 -> Data Type Conversion2/1
  Add1/1 -> Memory1/1, Gain1/1
  Memory1/1 -> Add1/2
  Relational Operator2/1 -> Data Type Conversion1/1
  Memory2/1 -> Add2/2
  Add2/1 -> Gain2/1, Memory2/1
  Relational Operator3/1 -> Data Type Conversion/1
  Memory3/1 -> Add3/2
  Add3/1 -> Memory3/1, Gain3/1
  Data Type Conversion/1 -> Add3/1
  Data Type Conversion1/1 -> Add2/1
  Data Type Conversion2/1 -> Add1/1
  Data Type Conversion3/1 -> Add/1
  vx/1 -> Compare To Constant6/1
  Compare To Constant6/1 -> AND4/1
  [lamda4] -> Compare To Constant10/1
  [lamda3] -> Compare To Constant9/1
  [lamda2] -> Compare To Constant8/1
  [lamda1] -> Compare To Constant7/1
  Compare To Constant7/1 -> Mux/1
  Compare To Constant8/1 -> Mux/2
  Compare To Constant9/1 -> Mux/3
  Compare To Constant10/1 -> Mux/4
  Mux/1 -> AND4/2
  AND4/1 -> Scope/1
  ? -> Abs/1
  Abs/1 -> Compare To Constant11/1
  Compare To Constant11/1 -> AND8/2, AND7/2, AND6/2, AND5/2
  AND/1 -> AND5/1
  AND1/1 -> AND6/1
  AND2/1 -> AND7/1
  AND3/1 -> AND8/1
  [lamda1] -> FL/1(lamda)
  Demux3/1 -> FL/2(Tload_hat)
  Sum5/1 -> Demux3/1, Compare To Constant4/1, Scope22/1
  az/1 -> Scope1/1, RR/3(az), RL/3(az), FR/3(az), FL/3(az)
  FL/1(airborne_flag) -> Scope6/2, Scope2/1
  FL/2(confidence) -> Scope2/2
  [lamda2] -> FR/1(lamda)
  [lamda3] -> RL/1(lamda)
  [lamda4] -> RR/1(lamda)
  Demux3/2 -> RR/2(Tload_hat), RL/2(Tload_hat), FR/2(Tload_hat)
  Demux1/2 -> FR/4(domega), Gain19/1
  Demux1/3 -> RL/4(domega), Gain18/1
  Demux1/4 -> RR/4(domega), Gain20/1
  FR/1(airborne_flag) -> Scope3/1
  FR/2(confidence) -> Scope3/2
  RL/1(airborne_flag) -> Scope4/1
  RL/2(confidence) -> Scope4/2
  RR/1(airborne_flag) -> Scope5/1
  RR/2(confidence) -> Scope5/2

== system tractor_mu/软土分配策略 ==
  sp_all : Inport
  vx(m/s) : Inport  Port=2
  st : Inport  Port=3
  Tmax : Inport  Port=4
  base_Torque : Inport  Port=5
  Constant : Constant  OutDataTypeStr=single
  Data Type Conversion : DataTypeConversion  OutDataTypeStr=single  SaturateOnIntegerOverflow=off  RndMeth=Floor
  Data Type Conversion1 : DataTypeConversion  OutDataTypeStr=single  SaturateOnIntegerOverflow=off  RndMeth=Floor
  Demux : Demux
  Gain : Gain  Gain=0.8  OutDataTypeStr=single
  MATLAB Function : MATLAB Function  TreatAsAtomicUnit=on
  MATLAB Function1 : MATLAB Function  TreatAsAtomicUnit=on
  Mux : Mux
  Mux1 : Mux
  Unit Delay : UnitDelay  SampleTime=-1  HasFrameUpgradeWarning=on
  Tfl_soft : Outport
  Tfr_soft : Outport  Port=2
  Trl_soft : Outport  Port=3
  Trr_soft : Outport  Port=4
  wires:
  vx(m/s)/1 -> MATLAB Function/3(longitudinal_speed_mps)
  st/1 -> MATLAB Function/2(front_steer_angles_deg)
  sp_all/1 -> Data Type Conversion/1
  Data Type Conversion/1 -> MATLAB Function/1(wheel_speeds_rpm)
  Constant/1 -> MATLAB Function/5(drive_torque_enabled)
  base_Torque/1 -> MATLAB Function1/2(baseline_torques_n_m), MATLAB Function/6(baseline_torques_n_m)
  Tmax/1 -> MATLAB Function1/3(wheel_torque_limits_n_m), Gain/1
  Gain/1 -> MATLAB Function/7(wheel_torque_limits_n_m)
  MATLAB Function/1(selected_torques_n_m) -> Data Type Conversion1/1
  Unit Delay/1 -> MATLAB Function/4(applied_torques_n_m)
  Data Type Conversion1/1 -> Unit Delay/1  "Tfl_soft"
  Demux/1 -> Tfl_soft/1
  Demux/2 -> Tfr_soft/1
  Demux/3 -> Trl_soft/1
  Demux/4 -> Trr_soft/1
  [lamda1] -> Mux/1
  [lamda2] -> Mux/2
  [lamda4] -> Mux/4
  [lamda3] -> Mux/3
  Mux/1 -> MATLAB Function1/1(measured_kappa)
  MATLAB Function1/1(torque_l1_n_m) -> Mux1/1
  MATLAB Function1/2(torque_r1_n_m) -> Mux1/2
  MATLAB Function1/3(torque_l2_n_m) -> Mux1/3
  MATLAB Function1/4(torque_r2_n_m) -> Mux1/4
  Mux1/1 -> Demux/1

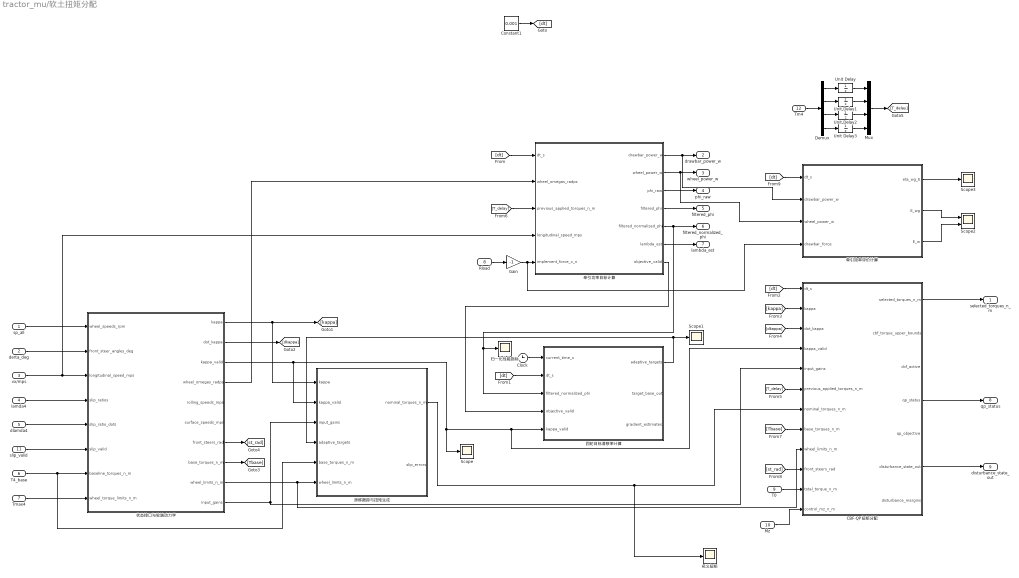
== system tractor_mu/软土扭矩分配 ==
  sp_all : Inport
  derta_deg : Inport  Port=2
  vx/mps : Inport  Port=3
  lamda4 : Inport  Port=4
  dlamda4 : Inport  Port=5
  T4_base : Inport  Port=6
  Tmax4 : Inport  Port=7
  Rload : Inport  Port=8
  T0 : Inport  Port=9
  Mz : Inport  Port=10
  slip_valid : Inport  Port=11
  Tm4 : Inport  Port=12
  CBF-QP扭矩分配 : MATLAB Function  TreatAsAtomicUnit=on
  Clock : Clock
  Constant1 : Constant  Value=0.001
  Demux : Demux
  Gain : Gain  Gain=-1
  Mux : Mux
  Scope : Scope
  Scope1 : Scope
  Scope2 : Scope  NumInputPorts=2
  Scope3 : Scope
  Unit Delay{,1..3} (4 alike) : UnitDelay  SampleTime=-1  HasFrameUpgradeWarning=on
  名义扭矩 : Scope
  四轮目标滑移率计算 : MATLAB Function  TreatAsAtomicUnit=on
  归一化性能指标 : Scope
  滑移跟踪与扭矩生成 : MATLAB Function  TreatAsAtomicUnit=on
  牵引功率目标计算 : MATLAB Function  TreatAsAtomicUnit=on
  牵引效率评价计算 : MATLAB Function  TreatAsAtomicUnit=on
  状态接口与轮端动力学 : MATLAB Function  TreatAsAtomicUnit=on
  selected_torques_n_m : Outport
  drawbar_power_w : Outport  Port=2
  wheel_power_w : Outport  Port=3
  phi_raw : Outport  Port=4
  filtered_phi : Outport  Port=5
  filtered_normalized_phi : Outport  Port=6
  lambda_est : Outport  Port=7
  qp_status : Outport  Port=8
  disturbance_state_out : Outport  Port=9
  wires:
  sp_all/1 -> 状态接口与轮端动力学/1(wheel_speeds_rpm)
  derta_deg/1 -> 状态接口与轮端动力学/2(front_steer_angles_deg)
  vx/mps/1 -> 牵引功率目标计算/4(longitudinal_speed_mps), 状态接口与轮端动力学/3(longitudinal_speed_mps)
  lamda4/1 -> 状态接口与轮端动力学/4(slip_ratios)
  dlamda4/1 -> 状态接口与轮端动力学/5(slip_ratio_dots)
  slip_valid/1 -> 状态接口与轮端动力学/6(slip_valid)
  T4_base/1 -> 滑移跟踪与扭矩生成/5(base_torques_n_m), 状态接口与轮端动力学/7(baseline_torques_n_m)
  Tmax4/1 -> 状态接口与轮端动力学/8(wheel_torque_limits_n_m)
  [dt] -> 牵引功率目标计算/1(dt_s)
  状态接口与轮端动力学/4(wheel_omegas_radps) -> 牵引功率目标计算/2(wheel_omegas_radps)
  [T_delay] -> 牵引功率目标计算/3(previous_applied_torques_n_m)
  Rload/1 -> Gain/1
  Clock/1 -> 四轮目标滑移率计算/1(current_time_s)
  Constant1/1 -> [dt]
  [dt] -> 四轮目标滑移率计算/2(dt_s)
  牵引功率目标计算/5(filtered_normalized_phi) -> filtered_normalized_phi/1, 归一化性能指标/1, 四轮目标滑移率计算/3(filtered_normalized_phi)
  状态接口与轮端动力学/3(kappa_valid) -> 滑移跟踪与扭矩生成/2(kappa_valid), Scope/1, CBF-QP扭矩分配/4(kappa_valid), 四轮目标滑移率计算/5(kappa_valid)
  牵引功率目标计算/7(objective_valid) -> 四轮目标滑移率计算/4(objective_valid)
  状态接口与轮端动力学/1(kappa) -> [kappa], 滑移跟踪与扭矩生成/1(kappa)
  状态接口与轮端动力学/10(input_gains) -> CBF-QP扭矩分配/5(input_gains), 滑移跟踪与扭矩生成/3(input_gains)
  四轮目标滑移率计算/1(adaptive_targets) -> Scope1/1, 滑移跟踪与扭矩生成/4(adaptive_targets)
  状态接口与轮端动力学/9(wheel_limits_n_m) -> CBF-QP扭矩分配/9(wheel_limits_n_m), 滑移跟踪与扭矩生成/6(wheel_limits_n_m)
  [dt] -> CBF-QP扭矩分配/1(dt_s)
  [kappa] -> CBF-QP扭矩分配/2(kappa)
  状态接口与轮端动力学/2(dot_kappa) -> [dkappa]
  [dkappa] -> CBF-QP扭矩分配/3(dot_kappa)
  [T_delay] -> CBF-QP扭矩分配/6(previous_applied_torques_n_m)
  滑移跟踪与扭矩生成/1(nominal_torques_n_m) -> 名义扭矩/1, CBF-QP扭矩分配/7(nominal_torques_n_m)
  状态接口与轮端动力学/8(base_torques_n_m) -> [Tbase]
  [Tbase] -> CBF-QP扭矩分配/8(base_torques_n_m)
  状态接口与轮端动力学/7(front_steers_rad) -> [st_rad]
  [st_rad] -> CBF-QP扭矩分配/10(front_steers_rad)
  T0/1 -> CBF-QP扭矩分配/11(total_torque_n_m)
  Mz/1 -> CBF-QP扭矩分配/12(control_mz_n_m)
  CBF-QP扭矩分配/1(selected_torques_n_m) -> selected_torques_n_m/1
  牵引功率目标计算/1(drawbar_power_w) -> 牵引效率评价计算/2(drawbar_power_w), drawbar_power_w/1
  牵引功率目标计算/2(wheel_power_w) -> 牵引效率评价计算/3(wheel_power_w), wheel_power_w/1
  牵引功率目标计算/3(phi_raw) -> phi_raw/1
  牵引功率目标计算/4(filtered_phi) -> filtered_phi/1
  牵引功率目标计算/6(lambda_est) -> lambda_est/1
  CBF-QP扭矩分配/4(qp_status) -> qp_status/1
  CBF-QP扭矩分配/6(disturbance_state_out) -> disturbance_state_out/1
  Demux/1 -> Unit Delay/1
  Demux/2 -> Unit Delay1/1
  Demux/3 -> Unit Delay2/1
  Demux/4 -> Unit Delay3/1
  Unit Delay/1 -> Mux/1
  Unit Delay1/1 -> Mux/2
  Unit Delay2/1 -> Mux/3
  Unit Delay3/1 -> Mux/4
  Mux/1 -> [T_delay]
  Tm4/1 -> Demux/1
  [dt] -> 牵引效率评价计算/1(dt_s)
  Gain/1 -> 牵引效率评价计算/4(drawbar_force), 牵引功率目标计算/5(implement_force_x_n)
  牵引效率评价计算/2(E_wg) -> Scope2/1
  牵引效率评价计算/3(E_w) -> Scope2/2
  牵引效率评价计算/1(eta_wg_E) -> Scope3/1

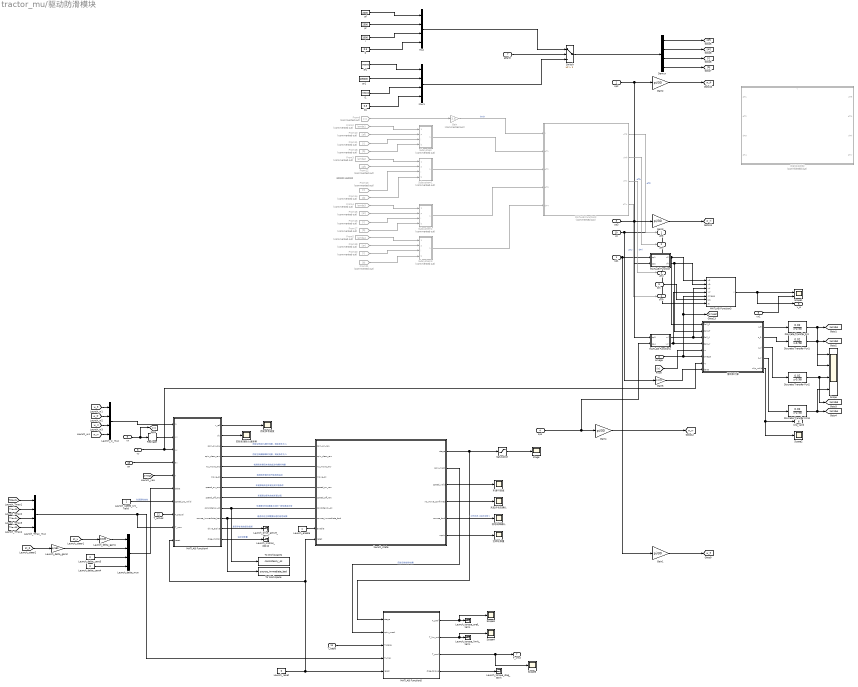
== system tractor_mu/驱动防滑模块 ==
  note: 300000
      | 450000
  sp1 : Inport
  sp2 : Inport  Port=2
  sp3 : Inport  Port=3
  sp4 : Inport  Port=4
  vx : Inport  Port=5
  vy : Inport  Port=6
  gearD : Inport  Port=7
  omega : Inport  Port=8
  brk : Inport  Port=9
  st : Inport  Port=10
  T_base : Inport  Port=11
  T_actual : Inport  Port=12
  ax : Inport  Port=13
  Demux : Demux
  Discrete Transfer Fcn{,1..3} (4 alike) : DiscreteTransferFcn  Numerator=[0.02]  Denominator=[1 -0.98]
  From10 : From  Commented=on  GotoTag=pf
  From{11,13,16,20} (4 alike) : From  Commented=on  GotoTag=i
  From12 : From  Commented=on  GotoTag=pf
  From{14,17..18,21} (4 alike) : From  Commented=on  GotoTag=b
  From15 : From  Commented=on  GotoTag=pr
  From19 : From  Commented=on  GotoTag=pr
  From2 : From  Commented=on  GotoTag=lamda1  TagVisibility=global
  From3 : From  Commented=on  GotoTag=lamda2  TagVisibility=global
  From4 : From  Commented=on  GotoTag=lamda3  TagVisibility=global
  From5 : From  Commented=on  GotoTag=lamda4  TagVisibility=global
  From6 : From  Commented=on  GotoTag=v
  Gain : Gain  Commented=on  Gain=3.6
  Gain{1..4} (4 alike) : Gain  Gain=pi/30
  Gain5 : Gain  Gain=pi/180
  Launch_Tmax_mux : Mux
  Launch_delta_gain1 : Gain  Gain=pi/180
  Launch_delta_gain2 : Gain  Gain=pi/180
  Launch_delta_mux : Mux
  Launch_delta_zero3 : Constant  Value=0
  Launch_delta_zero4 : Constant  Value=0
  Launch_drive_active_term : Terminator
  Launch_enable : Constant
  Launch_motion_obs12 : Terminator
  Launch_reset : Constant  Value=0
  Launch_speed_src_valid : Constant
  Launch_torque_diag_term : Terminator
  Launch_torque_limit_term : Terminator
  Launch_torque_pref_term : Terminator
  Launch_w_mux : Mux
  MATLAB Function : MATLAB Function  TreatAsAtomicUnit=on
  MATLAB Function1 : MATLAB Function  TreatAsAtomicUnit=on
  MATLAB Function2 : MATLAB Function  Commented=on  TreatAsAtomicUnit=on
  MATLAB Function3 : MATLAB Function  TreatAsAtomicUnit=on
  MATLAB Function4 : MATLAB Function  TreatAsAtomicUnit=on
  MATLAB Function5 : MATLAB Function  TreatAsAtomicUnit=on
  Mux : Mux
  Mux1 : Mux
  Reshape : Reshape  OutputDimensionality=Customize  OutputDimensions=[1 1]
  Saturation : Saturate  UpperLimit=10  LowerLimit=0
  Scope : Scope  NumInputPorts=4
  Scope1 : Scope  NumInputPorts=2
  Scope{2..5} (4 alike) : Scope
  Subsystem : Subsystem  Commented=on
  Subsystem1 : Subsystem  Commented=on
  Subsystem2 : Subsystem  Commented=on
  Subsystem3 : Subsystem  Commented=on
  Switch : Switch  Criteria=u2 > Threshold  Threshold=1  SaturateOnIntegerOverflow=off  InputSameDT=off
  To Workspace : ToWorkspace  VariableName=source_immediate_bad  SaveFormat=Structure With Time  SampleTime=-1
  To Workspace1 : ToWorkspace  VariableName=consistency_ok  SaveFormat=Structure With Time  SampleTime=-1
  b : Constant  Value=0.3
  b1 : Constant  Value=0.3
  i : Constant  Value=2000
  i1 : Constant  Value=35000
  launch_state : Stateflow chart  TreatAsAtomicUnit=on
  pf : Constant  Value=2000
  pf1 : Constant  Value=90000
  pr : Constant  Value=2500
  pr1 : Constant  Value=105000
  stage : Scope
  vx1 : InportShadow  Port=5
  信号故障确认 : Scope
  四轮参考速度 : Scope
  四轮轮端轮心速度差 : Scope
  未起步状态确认 : Scope
  滑转率计算 : Subsystem
  空转轮数量 : Scope
  车速可信度 : Scope
  转矩协调控制 : Stateflow chart  Commented=on  TreatAsAtomicUnit=on
      settings: PortSchema="{\"entries\":[{\"content\":{\"sides\":[{\"content\":{\"connectorIds\":[\"In2\",\"In3\",\"In4\",\"In5\"]},\"type\":\"ConnectorPlacement.EquallySpacedRectSide\",\"uuid\":\"973a9b84-73ad-47b8-a26a-d7aec675acf5\"},{\"content\":{\"connectorIds\":[\"Out1\",\"Out2\",\"Out3\",\"Out4\"],\"side\":\"RIGHT\"},\"type\":\"ConnectorPlacement.EquallySpacedRectSide\",\"uuid\":\"de1e0d9b-25bd-4ac7-be2f-c0268a60ba4f\"},{\"content\":{\"connectorIds\":[\"In1\"],\"side\":\"TOP\"},\"type\":\"ConnectorPlacement.EquallySpacedRectSide\",\"uuid\":\"9ce864d3-2ff1-442a-967b-03df7267dcea\"}]},\"type\":\"ConnectorPlacement.EquallySpacedConnector\",\"uuid\":\"50a94803-c5b1-4606-ba3c-9c5c7d907f69\"}],\"packageUris\":[\"http://schema.mathworks.com/mf0/Connector/R2020b\"],\"version\":\"1.0\"}"
  dTfl : Outport
  dTfr : Outport  Port=2
  dTrl : Outport  Port=3
  dTrr : Outport  Port=4
  v_e : Outport  Port=5
  slip_valid : Outport  Port=6
  T_cmd : Outport  Port=7
  tag scope: lamda1=global, lamda2=global, lamda3=global, lamda4=global, w_fl=global, w_fr=global, w_rl=global, w_rr=global
  wires:
  [w_fl] -> Launch_w_mux/1
  pf/1 -> Mux/1
  pr/1 -> Mux/2
  i/1 -> Mux/3
  [st_R] -> Launch_delta_gain2/1
  b/1 -> Mux/4
  [TMaxRL] -> Launch_Tmax_mux/3
  pf1/1 -> Mux1/1
  pr1/1 -> Mux1/2
  Mux1/1 -> Switch/3
  Subsystem/1(dT1) -> MATLAB Function2/2(dT1)
  i1/1 -> Mux1/3
  b1/1 -> Mux1/4
  launch_state/6(nspin) -> 空转轮数量/1
  From6/1 -> Gain/1
  From2/1 -> Subsystem/1(lamda1)
  From10/1 -> Subsystem/2(p)
  Subsystem3/1(dT1) -> MATLAB Function2/5(dT4)
  From11/1 -> Subsystem/3(i)
  [w_fr] -> Launch_w_mux/2
  From18/1 -> Subsystem/4(b)
  Launch_Tmax_mux/1 -> MATLAB Function4/9(T_max), MATLAB Function5/4(T_max)
  From4/1 -> Subsystem2/1(lamda3)
  From3/1 -> Subsystem1/1(lamda2)
  From12/1 -> Subsystem1/2(p)
  From14/1 -> Subsystem1/4(b)
  From13/1 -> Subsystem1/3(i)
  sp1/1 -> MATLAB Function/1(sp1), Gain1/1
  From15/1 -> Subsystem2/2(p)
  MATLAB Function2/4(dTrr) -> dTrr/1  "dTrr"
  From16/1 -> Subsystem2/3(i)
  MATLAB Function5/2(T_lim_out) -> Scope4/1, Launch_torque_limit_term/1
  Launch_enable/1 -> launch_state/9(enable)
  From17/1 -> Subsystem2/4(b)
  From5/1 -> Subsystem3/1(lamda4)
  From21/1 -> Subsystem3/4(b)
  From19/1 -> Subsystem3/2(p)
  [st_L] -> Launch_delta_gain1/1
  From20/1 -> Subsystem3/3(i)
  Launch_reset/1 -> MATLAB Function5/5(reset), launch_state/10(reset), MATLAB Function4/10(reset)
  [TMaxFL] -> Launch_Tmax_mux/1
  st/1 -> MATLAB Function3/7(st), Gain5/1
  [TMaxFR] -> Launch_Tmax_mux/2
  [TMaxRR] -> Launch_Tmax_mux/4
  Mux/1 -> Switch/1
  gearD/1 -> Switch/2
  MATLAB Function2/1(dTfl) -> dTfl/1  "dTfl"
  Launch_w_mux/1 -> MATLAB Function4/1(w)
  launch_state/1(stage) -> Saturation/1, MATLAB Function5/1(stage)  "工作状态（起步过程）"
  Gain/1 -> MATLAB Function2/1(v)  "km/h"
  Subsystem1/1(dT1) -> MATLAB Function2/3(dT2)
  [w_rl] -> Launch_w_mux/3
  launch_state/2(spin_mask) -> MATLAB Function5/2(spin_mask)  "四轮空转锁存结果"
  Subsystem2/1(dT1) -> MATLAB Function2/4(dT3)
  launch_state/3(speed_valid) -> 车速可信度/1
  launch_state/4(no_move_confirmed) -> 未起步状态确认/1
  launch_state/5(source_bad) -> 信号故障确认/1
  T_base/1 -> MATLAB Function5/3(T_base)
  MATLAB Function5/1(T_pref) -> Scope3/1, Launch_torque_pref_term/1
  Switch/1 -> Demux/1
  sp2/1 -> MATLAB Function/2(sp2), Gain2/1
  MATLAB Function2/2(dTfr) -> dTfr/1  "dTfr"
  MATLAB Function2/3(dTrl) -> dTrl/1  "dTrl"
  ax/1 -> MATLAB Function4/4(ax)
  sp3/1 -> MATLAB Function1/1(sp3), Gain3/1
  Gain2/1 -> [w_fr]
  MATLAB Function5/3(T_cmd) -> Scope5/1, T_cmd/1
  MATLAB Function5/4(diag_torque) -> Launch_torque_diag_term/1
  sp4/1 -> MATLAB Function1/2(sp4), Gain4/1
  [w_rr] -> Launch_w_mux/4
  Launch_delta_gain1/1 -> Launch_delta_mux/1
  Launch_delta_gain2/1 -> Launch_delta_mux/2
  Launch_delta_zero3/1 -> Launch_delta_mux/3
  Launch_delta_zero4/1 -> Launch_delta_mux/4
  Demux/1 -> [pf]
  Demux/2 -> [pr]
  滑转率计算/4(s_rr) -> Discrete Transfer Fcn3/1
  Demux/3 -> [i]
  Demux/4 -> [b]
  Gain3/1 -> [w_rl]
  MATLAB Function/1(vfl) -> MATLAB Function3/1(vfl), 滑转率计算/1(Roll_fl)
  MATLAB Function/2(vfr) -> MATLAB Function3/2(vfr), 滑转率计算/2(Roll_fr)
  brk/1 -> MATLAB Function3/6(brk)
  MATLAB Function1/1(vrl) -> MATLAB Function3/3(vrl), 滑转率计算/3(Roll_rl)
  MATLAB Function1/2(vrr) -> MATLAB Function3/4(vrr), 滑转率计算/4(Roll_rr)
  omega/1 -> [omega], MATLAB Function3/5(omega), 滑转率计算/6(omega)
  [v] -> 滑转率计算/5(vx)
  Gain5/1 -> 滑转率计算/8(derta)
  vy/1 -> 滑转率计算/7(vy), MATLAB Function4/3(vy)
  vx/1 -> [v], Reshape/1
  Gain1/1 -> [w_fl]
  [omega] -> MATLAB Function4/5(r)
  Launch_delta_mux/1 -> MATLAB Function4/6(delta)
  Launch_speed_src_valid/1 -> MATLAB Function4/7(speed_src_valid)  "车速源有效性"
  Gain4/1 -> [w_rr]
  MATLAB Function3/1(v) -> Scope1/1, v_e/1
  vx1/1 -> Scope1/2
  滑转率计算/1(s_fl) -> Discrete Transfer Fcn/1
  滑转率计算/2(s_fr) -> Discrete Transfer Fcn1/1
  滑转率计算/3(s_rl) -> Discrete Transfer Fcn2/1
  滑转率计算/5(slip_valid) -> slip_valid/1, Scope2/1
  MATLAB Function4/1(v_ref) -> 四轮参考速度/1
  MATLAB Function4/2(dv) -> 四轮轮端轮心速度差/1
  MATLAB Function4/3(spin_on_raw) -> launch_state/1(spin_on_raw)  "四轮空转进入瞬时判据，满足条件为 1"
  MATLAB Function4/4(spin_clear_raw) -> launch_state/2(spin_clear_raw)  "四轮空转解除瞬时判据，满足条件为 1"
  MATLAB Function4/5(no_move_raw) -> launch_state/3(no_move_raw)  "检测到车辆仍未有效起步的瞬时判据"
  MATLAB Function4/6(move_ok) -> launch_state/4(move_ok)  "检测到车辆已经开始有效运动"
  MATLAB Function4/7(speed_on_raw) -> launch_state/5(speed_on_raw)  "车速源有效且车速达到可信条件"
  MATLAB Function4/8(speed_off_raw) -> launch_state/6(speed_off_raw)  "车速源立即失效或车速过低"
  MATLAB Function4/9(consistency_ok) -> To Workspace1/1, launch_state/7(consistency_ok)  "车速微分和加速度之间的一致性是否正常"
  MATLAB Function4/10(source_immediate_bad) -> To Workspace/1, launch_state/8(source_immediate_bad)  "是否存在立即需要处理的信号故障"
  MATLAB Function4/11(drive_active) -> Launch_drive_active_term/1  "是否存在有效驱动扭矩"
  MATLAB Function4/12(diag_motion) -> Launch_motion_obs12/1  "运动诊断量"
  Discrete Transfer Fcn/1 -> [lamda1], Scope/1
  Discrete Transfer Fcn1/1 -> Scope/2, [lamda2]
  Discrete Transfer Fcn2/1 -> Scope/3, [lamda3]
  Discrete Transfer Fcn3/1 -> Scope/4, [lamda4]
  Reshape/1 -> MATLAB Function4/2(vx)
  Saturation/1 -> stage/1
  T_actual/1 -> MATLAB Function4/8(T_actual)

== system tractor_mu/Dugoff轮胎模型/alpha_lamda ==
  vx : Inport
  vy : Inport  Port=2
  wz : Inport  Port=3
  delta_fl : Inport  Port=4
  delta_fr : Inport  Port=5
  w_fl : Inport  Port=6
  w_fr : Inport  Port=7
  w_rl : Inport  Port=8
  w_rr : Inport  Port=9
  Scope : Scope  NumInputPorts=4
  alpha : Subsystem
  lamda : Subsystem
  lamda_fl : Outport
  lamda_fr : Outport  Port=2
  lamda_rl : Outport  Port=3
  lamda_rr : Outport  Port=4
  alpha_fl : Outport  Port=5
  alpha_fr : Outport  Port=6
  alpha_rl : Outport  Port=7
  alpha_rr : Outport  Port=8
  wires:
  lamda/3(lamda_rl) -> Scope/3, lamda_rl/1
  lamda/4(lamda_rr) -> Scope/4, lamda_rr/1
  lamda/2(lamda_fr) -> Scope/2, lamda_fr/1
  lamda/1(lamda_fl) -> Scope/1, lamda_fl/1
  w_rr/1 -> lamda/9(w_rr)
  w_rl/1 -> lamda/8(w_rl)
  w_fr/1 -> lamda/7(w_fr)
  w_fl/1 -> lamda/6(w_fl)
  delta_fr/1 -> alpha/5(delta_fr), lamda/5(delta_fr)
  delta_fl/1 -> alpha/4(delta_fl), lamda/4(delta_fl)
  wz/1 -> alpha/3(wz), lamda/3(wz)
  vy/1 -> alpha/2(vy), lamda/2(vy)
  vx/1 -> alpha/1(vx), lamda/1(vx)
  alpha/4(alpha_rr) -> alpha_rr/1
  alpha/3(alpha_rl) -> alpha_rl/1
  alpha/2(alpha_fr) -> alpha_fr/1
  alpha/1(alpha_fl) -> alpha_fl/1
